simulink model "thermostat_sf"  (R2026b)
settings: Solver=ode3  StopTime=400  FixedStep=0.1
undefined symbols (not defined in the file): SOChigh, SOClow
settings Model: Creator=Hamza  LastModifiedBy=Hamza

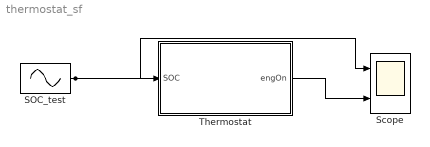
== system thermostat_sf ==
  SOC_test : Sin  Amplitude=0.175  Bias=0.575  Frequency=2*pi/200  SampleTime=0
  Scope : Scope  NumInputPorts=2
  Thermostat : Stateflow chart  TreatAsAtomicUnit=on
  wires:
  SOC_test/1 -> Thermostat/1(SOC), Scope/1
  Thermostat/1(engOn) -> Scope/2

== stateflow chart thermostat_sf/Thermostat ==
  settings: updateMethod=DISCRETE  sampleTime=0.1
  state Engine_OFF
    entry: engOn = 0;
  state Engine_ON
    entry: engOn = 1;
  Engine_ON -> Engine_OFF : [SOC > SOChigh]
  (default) -> Engine_OFF
  Engine_OFF -> Engine_ON : [SOC < SOClow]
  data: SOC input; engOn output; SOClow parameter; SOChigh parameter
